simulink subsystem "lla2Pos"  (R2026a)
settings: Solver=VariableStepAuto
values from neighbouring files (symbols this model uses):
  gpsConversion = 6391803.4646718353    [navParams.sldd]
libraries: simulink_extras x3
settings Model: Creator=maxhu  LastModifiedBy=maxhu

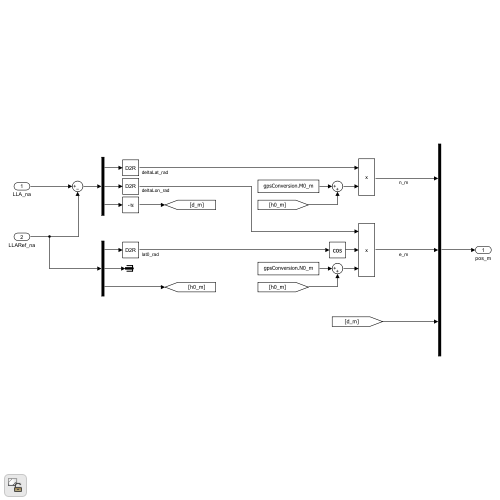
[thumbnail: Simulink's stored preview of the top-level diagram]
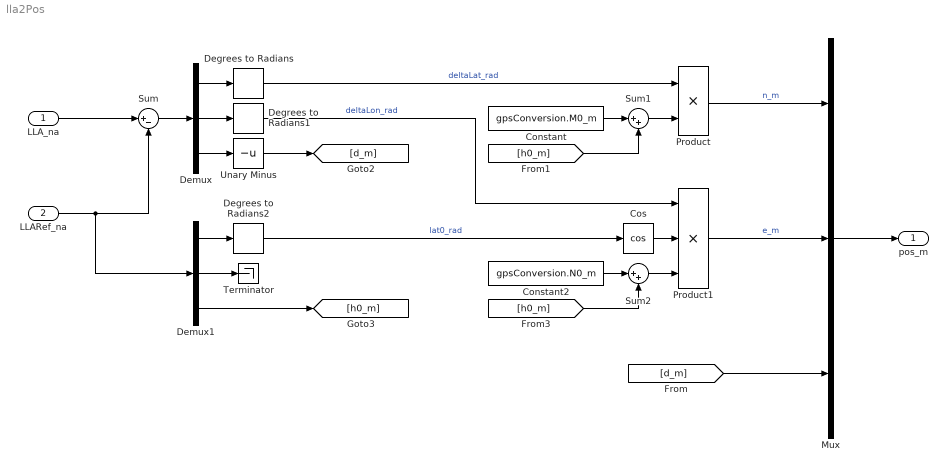
== system lla2Pos ==
  LLA_na : Inport
  LLARef_na : Inport  Port=2
  Constant : Constant  Value=gpsConversion.M0_m
  Constant2 : Constant  Value=gpsConversion.N0_m
  Cos : Trigonometry  Operator=cos
  Degrees to Radians : simulink_extras/Transformations/Degrees to Radians
  Degrees to Radians1 : simulink_extras/Transformations/Degrees to Radians
  Degrees to Radians2 : simulink_extras/Transformations/Degrees to Radians
  Demux : Demux  Outputs=3
  Demux1 : Demux  Outputs=3
  Mux : Mux  Inputs=3
  Product : Product
  Product1 : Product  Inputs=3
  Sum : Sum  Inputs=|+-
  Sum1 : Sum  Inputs=|++
  Sum2 : Sum  Inputs=|++
  Terminator : Terminator
  Unary Minus : UnaryMinus
  pos_m : Outport
  wires:
  LLA_na/1 -> Sum/1
  LLARef_na/1 -> Sum/2, Demux1/1
  Sum/1 -> Demux/1
  Demux/1 -> Degrees to Radians/1
  Demux/2 -> Degrees to Radians1/1
  Degrees to Radians/1 -> Product/1  "deltaLat_rad"
  Demux/3 -> Unary Minus/1
  Unary Minus/1 -> [d_m]
  Demux1/3 -> [h0_m]
  Constant/1 -> Sum1/1
  Sum1/1 -> Product/2
  [h0_m] -> Sum1/2
  Degrees to Radians1/1 -> Product1/1  "deltaLon_rad"
  Constant2/1 -> Sum2/1
  [h0_m] -> Sum2/2
  Sum2/1 -> Product1/3
  Demux1/2 -> Terminator/1
  Demux1/1 -> Degrees to Radians2/1
  Cos/1 -> Product1/2
  Degrees to Radians2/1 -> Cos/1  "lat0_rad"
  Product/1 -> Mux/1  "n_m"
  Product1/1 -> Mux/2  "e_m"
  [d_m] -> Mux/3
  Mux/1 -> pos_m/1
